simulink model "EV_BMS_ISO26262_Model"  (R2024b)
settings: Solver=ode4  StartTime=0.0  StopTime=600.0  FixedStep=0.1  RelTol=1e-3
PreLoadFcn:
  | bms_params = init_bms_parameters(); wltp_cycle = generate_drive_cycles('WLTP', 600, 0.1); I_drive_series = timeseries(wltp_cycle.current, wltp_cycle.time);
InitFcn:
  | bms_params = init_bms_parameters(); wltp_cycle = generate_drive_cycles('WLTP', 600, 0.1); I_drive_series = timeseries(wltp_cycle.current, wltp_cycle.time);
settings Model: Creator=us  LastModifiedBy=us

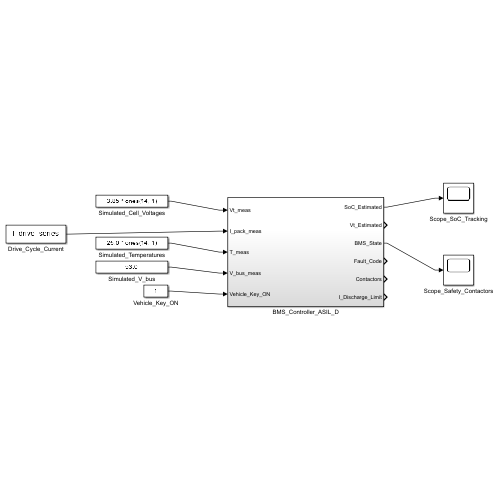
[thumbnail: Simulink's stored preview of the top-level diagram]
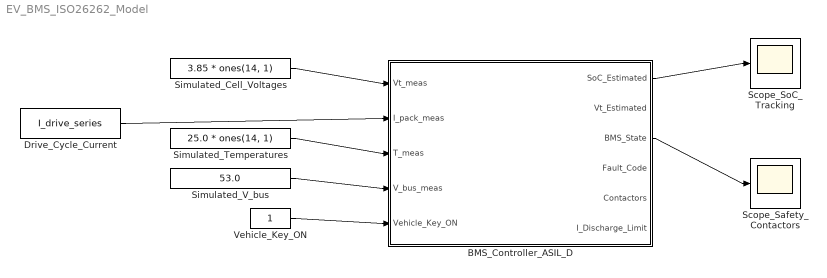
== system EV_BMS_ISO26262_Model ==
  BMS_Controller_ASIL_D : Subsystem
  Drive_Cycle_Current : FromWorkspace  VariableName=I_drive_series
  Scope_Safety_Contactors : Scope
  Scope_SoC_Tracking : Scope
  Simulated_Cell_Voltages : Constant  Value=3.85 * ones(14, 1)
  Simulated_Temperatures : Constant  Value=25.0 * ones(14, 1)
  Simulated_V_bus : Constant  Value=53.0
  Vehicle_Key_ON : Constant
  wires:
  BMS_Controller_ASIL_D/1(SoC_Estimated) -> Scope_SoC_Tracking/1
  BMS_Controller_ASIL_D/3(BMS_State) -> Scope_Safety_Contactors/1
  Vehicle_Key_ON/1 -> BMS_Controller_ASIL_D/5(Vehicle_Key_ON)
  Drive_Cycle_Current/1 -> BMS_Controller_ASIL_D/2(I_pack_meas)
  Simulated_Cell_Voltages/1 -> BMS_Controller_ASIL_D/1(Vt_meas)
  Simulated_Temperatures/1 -> BMS_Controller_ASIL_D/3(T_meas)
  Simulated_V_bus/1 -> BMS_Controller_ASIL_D/4(V_bus_meas)

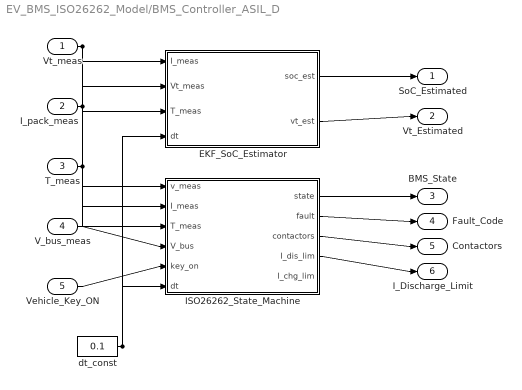
== system EV_BMS_ISO26262_Model/BMS_Controller_ASIL_D ==
  Vt_meas : Inport
  I_pack_meas : Inport  Port=2
  T_meas : Inport  Port=3
  V_bus_meas : Inport  Port=4
  Vehicle_Key_ON : Inport  Port=5
  EKF_SoC_Estimator : MATLAB Function  TreatAsAtomicUnit=on
  ISO26262_State_Machine : MATLAB Function  TreatAsAtomicUnit=on
  dt_const : Constant  Value=0.1
  SoC_Estimated : Outport
  Vt_Estimated : Outport  Port=2
  BMS_State : Outport  Port=3
  Fault_Code : Outport  Port=4
  Contactors : Outport  Port=5
  I_Discharge_Limit : Outport  Port=6
  wires:
  I_pack_meas/1 -> EKF_SoC_Estimator/1(I_meas), ISO26262_State_Machine/2(I_meas)
  Vt_meas/1 -> EKF_SoC_Estimator/2(Vt_meas), ISO26262_State_Machine/1(v_meas)
  T_meas/1 -> EKF_SoC_Estimator/3(T_meas), ISO26262_State_Machine/3(T_meas)
  dt_const/1 -> EKF_SoC_Estimator/4(dt), ISO26262_State_Machine/6(dt)
  EKF_SoC_Estimator/1(soc_est) -> SoC_Estimated/1
  EKF_SoC_Estimator/2(vt_est) -> Vt_Estimated/1
  V_bus_meas/1 -> ISO26262_State_Machine/4(V_bus)
  Vehicle_Key_ON/1 -> ISO26262_State_Machine/5(key_on)
  ISO26262_State_Machine/1(state) -> BMS_State/1
  ISO26262_State_Machine/2(fault) -> Fault_Code/1
  ISO26262_State_Machine/3(contactors) -> Contactors/1
  ISO26262_State_Machine/4(I_dis_lim) -> I_Discharge_Limit/1

== matlab function EV_BMS_ISO26262_Model/BMS_Controller_ASIL_D/ISO26262_State_Machine ==
  data: v_meas input; state output; I_meas input; T_meas input; V_bus input; key_on input; dt input; fault output; contactors output; I_dis_lim output; I_chg_lim output
function [state, fault, contactors, I_dis_lim, I_chg_lim] = ISO26262_State_Machine( ...
    v_meas, I_meas, T_meas, V_bus, key_on, dt)
state = 1;
fault = 0;
contactors = [0, 0, 0];
I_dis_lim = 0.0;
I_chg_lim = 0.0;
persistent bms_state fault_code precharge_timer
if isempty(bms_state)
    bms_state = 1;
    fault_code = 0;
    precharge_timer = 0.0;
end
v_max = max(v_meas); v_min = min(v_meas); t_max = max(T_meas); t_min = min(T_meas); v_sum = sum(v_meas);
if v_max >= 4.25, fault_code = 1;
elseif v_min <= 2.75, fault_code = 2;
elseif I_meas >= 120.0, fault_code = 3;
elseif I_meas <= -25.0, fault_code = 4;
elseif t_max >= 60.0, fault_code = 5;
elseif t_min <= -20.0, fault_code = 6;
end
if fault_code ~= 0
    bms_state = 6; contactors = [0, 0, 0]; I_dis_lim = 0.0; I_chg_lim = 0.0;
    state = bms_state; fault = fault_code; return;
end
switch bms_state
    case 1, bms_state = 2; contactors = [0, 0, 0];
    case 2
        contactors = [0, 0, 0];
        if V_bus > 10.0, bms_state = 6; fault_code = 8;
        elseif key_on >= 1, bms_state = 3; contactors = [0, 1, 1]; precharge_timer = 0.0; end
    case 3
        precharge_timer = precharge_timer + dt; contactors = [0, 1, 1];
        if V_bus >= 0.95 * v_sum, bms_state = 4; contactors = [1, 1, 0];
        elseif precharge_timer >= 0.500, bms_state = 6; fault_code = 7; contactors = [0, 0, 0]; end
    case {4, 5}
        if key_on == 0, bms_state = 2; contactors = [0, 0, 0];
        else
            if (t_max >= 45.0) || (t_min <= 5.0) || (v_max >= 4.20) || (v_min <= 3.00)
                bms_state = 5;
            else, bms_state = 4; end
            contactors = [1, 1, 0];
        end
    otherwise, bms_state = 6; contactors = [0, 0, 0];
end
if bms_state == 6, I_dis_lim = 0.0; I_chg_lim = 0.0;
elseif bms_state == 5, I_dis_lim = 40.0; I_chg_lim = 10.0;
else, I_dis_lim = 80.0; I_chg_lim = 20.0; end
state = bms_state; fault = fault_code;
end

== matlab function EV_BMS_ISO26262_Model/BMS_Controller_ASIL_D/EKF_SoC_Estimator ==
  data: I_meas input; soc_est output; Vt_meas input; T_meas input; dt input; vt_est output
function [soc_est, vt_est] = EKF_SoC_Estimator(I_meas, Vt_meas, T_meas, dt)
persistent x P
if isempty(x)
    x = [0.65; 0.0; 0.0];
    P = [0.20, 0, 0; 0, 0.01, 0; 0, 0, 0.01];
end
Q_n = 18000.0; R0_ref = 0.0150; R1 = 0.0085; C1 = 1500.0;
R2 = 0.0120; C2 = 6000.0; tau1 = R1 * C1; tau2 = R2 * C2;
alpha1 = exp(-dt / tau1); alpha2 = exp(-dt / tau2);
T_K = T_meas(1) + 273.15;
arrhenius = exp((22000.0 / 8.314) * (1.0 / T_K - 1.0 / 298.15));
R0 = R0_ref * arrhenius;
eta = 1.0;
if I_meas < 0, eta = 0.998; end
x_pred = [x(1) - (eta * dt / Q_n) * I_meas;
          alpha1 * x(2) + R1 * (1.0 - alpha1) * I_meas;
          alpha2 * x(3) + R2 * (1.0 - alpha2) * I_meas];
x_pred(1) = max(0.0, min(1.0, x_pred(1)));
Ad = [1.0, 0.0, 0.0; 0.0, alpha1, 0.0; 0.0, 0.0, alpha2];
Q_cov = diag([2.0e-6, 1.0e-5, 1.0e-5]);
P_pred = Ad * P * Ad' + Q_cov;
poly_c = [-1.94295, 8.52070, -18.71091, 21.62724, -12.16665, 3.71743, 3.15347];
s = x_pred(1);
Voc_pred = polyval(poly_c, s);
vt_est = Voc_pred - x_pred(2) - x_pred(3) - I_meas * R0;
dpoly_c = [-11.65770, 42.60350, -74.84364, 64.88172, -24.33330, 3.71743];
dVoc = max(0.05, polyval(dpoly_c, s));
C = [dVoc, -1.0, -1.0];
R_meas = 1.0e-3;
S = C * P_pred * C' + R_meas;
K = (P_pred * C') / S;
y_innov = Vt_meas(1) - vt_est;
x = x_pred + K * y_innov;
x(1) = max(0.0, min(1.0, x(1)));
IKC = eye(3) - K * C;
P = IKC * P_pred * IKC' + (K * R_meas) * K';
P = 0.5 * (P + P');
soc_est = x(1);
end
